simulink model "radial_fault_study_network"  (R2026b)
settings: Solver=ode23t  StopTime=0.15  MaxStep=5e-5
libraries: ee_lib x20, nesl_utility x8, simulink x5, simulink_extras x2, fl_lib x1
settings Model: Creator=ankes  LastModifiedBy=ankes
settings SimscapeCC: SimscapeLogType=all  SimscapeNominalValues="[{\"value\":\"1\",\"unit\":\"A\"},{\"value\":\"1\",\"unit\":\"bar\"},{\"value\":\"1\",\"unit\":\"cm^2\"},{\"value\":\"1\",\"unit\":\"cm^3/s\"},{\"value\":\"1\",\"unit\":\"kJ/kg\"},{\"value\":\"1\",\"unit\":\"kW\"},{\"value\":\"1\",\"unit\":\"l\"},{\"value\":\"1\",\"unit\":\"N\"},{\"value\":\"1\",\"unit\":\"N*m\"},{\"value\":\"1\",\"unit\":\"V\"},{\"value\":\"0.001\",\"unit\":\"Wb\"}]"  SimscapeUseEnergyAccounting=off

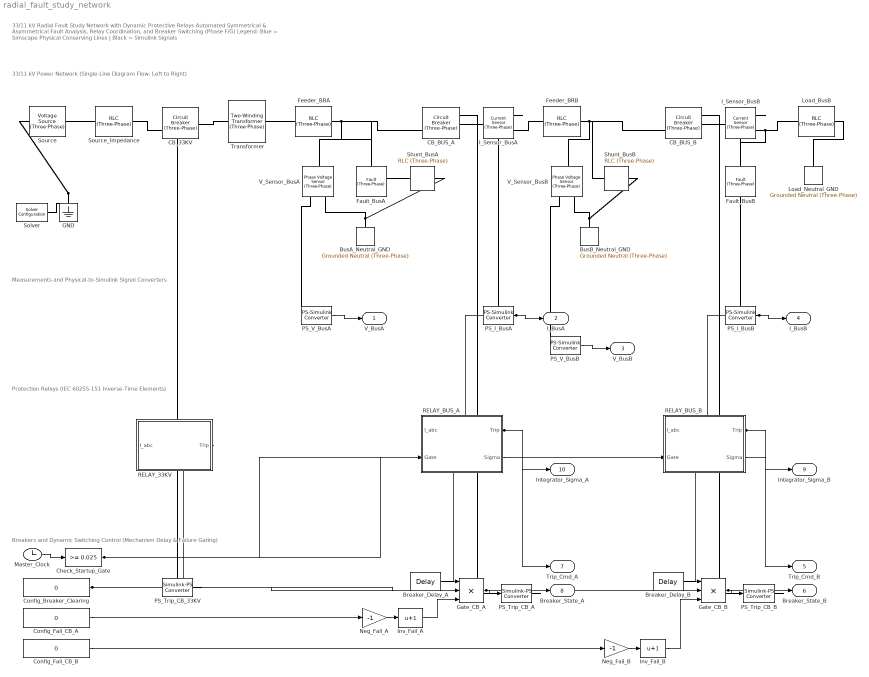
== system radial_fault_study_network ==
  note: 33/11 kV Radial Fault Study Network with Dynamic Protective Relays
      | Automated Symmetrical & Asymmetrical Fault Analysis, Relay Coordination, and Breaker Switching (Phase F/G)
      | Legend: Blue = Simscape Physical Conserving Lines  |  Black = Simulink Signals
  note: 33/11 kV Power Network (Single-Line Diagram Flow: Left to Right)
  note: Measurements and Physical-to-Simulink Signal Converters
  note: Protection Relays (IEC 60255-151 Inverse-Time Elements)
  note: Breakers and Dynamic Switching Control (Mechanism Delay & Failure Gating)
  Breaker_Delay_A : TransportDelay  DelayTime=0.06  BufferSize=8192
  Breaker_Delay_B : TransportDelay  DelayTime=0.05  BufferSize=8192
  BusA_Neutral_GND : ee_lib/Connectors & References/Grounded Neutral (Three-Phase)  port_option=ee.enum.threePhasePort.composite
  BusB_Neutral_GND : ee_lib/Connectors & References/Grounded Neutral (Three-Phase)  port_option=ee.enum.threePhasePort.composite
  CB_33KV : ee_lib/Switches & Breakers/Circuit Breaker (Three-Phase)  port_option=ee.enum.threePhasePort.composite  control_port_option=ee.enum.controlport.ps  R_closed=0.001 Ohm  G_open=1e-6 1/Ohm  threshold=0.5 V  breaker_behavior=ee.enum.switches.breakerBehavior.zeroCrossingEnable  i_th=1e-8 A
  CB_BUS_A : ee_lib/Switches & Breakers/Circuit Breaker (Three-Phase)  port_option=ee.enum.threePhasePort.composite  control_port_option=ee.enum.controlport.ps  R_closed=0.001 Ohm  G_open=1e-6 1/Ohm  threshold=0.5 V  breaker_behavior=ee.enum.switches.breakerBehavior.zeroCrossingEnable  i_th=1e-8 A
  CB_BUS_B : ee_lib/Switches & Breakers/Circuit Breaker (Three-Phase)  port_option=ee.enum.threePhasePort.composite  control_port_option=ee.enum.controlport.ps  R_closed=0.001 Ohm  G_open=1e-6 1/Ohm  threshold=0.5 V  breaker_behavior=ee.enum.switches.breakerBehavior.zeroCrossingEnable  i_th=1e-8 A
  Check_Startup_Gate : simulink/Logic and Bit Operations/Compare To Constant  relop=>=  const=0.025  OutDataTypeStr=boolean
  Config_Breaker_Clearing : Constant  Value=0
  Config_Fail_CB_A : Constant  Value=0
  Config_Fail_CB_B : Constant  Value=0
  Fault_BusA : ee_lib/Utilities/Fault (Three-Phase)  port_option=ee.enum.threePhasePort.composite  fault_type_option=ee.enum.fault_type_option.abc  R_pn_fault=0.001 Ohm  R_ng_fault=0.001 Ohm  exposemeasurement=ee.enum.exposemeasurement.hidden  enable_external_fault=ee.enum.external_fault.hidden  fault_threshold=0.5  fault_condition=ee.enum.fault_condition.fgt  fault_resettable=ee.enum.enable.no  enable_temporal_fault=ee.enum.enable.no  fault_start_time=999.0 s  fault_duration=0.20 s  G_parasitic=1e-4 1/Ohm  I_specify=off  I_priority=None  I=[0, 0, 0] A  I_nominal_specify=off  I_nominal_value=1  I_nominal_unit=A  i_ng_specify=off  i_ng_priority=None  i_ng=0 A  i_ng_nominal_specify=off  i_ng_nominal_value=1  i_ng_nominal_unit=A
  Fault_BusB : ee_lib/Utilities/Fault (Three-Phase)  port_option=ee.enum.threePhasePort.composite  fault_type_option=ee.enum.fault_type_option.abc  R_pn_fault=0.001 Ohm  R_ng_fault=0.001 Ohm  exposemeasurement=ee.enum.exposemeasurement.hidden  enable_external_fault=ee.enum.external_fault.hidden  fault_threshold=0.5  fault_condition=ee.enum.fault_condition.fgt  fault_resettable=ee.enum.enable.no  enable_temporal_fault=ee.enum.enable.yes  fault_start_time=0.05 s  fault_duration=0.20 s  G_parasitic=1e-4 1/Ohm  I_specify=off  I_priority=None  I=[0, 0, 0] A  I_nominal_specify=off  I_nominal_value=1  I_nominal_unit=A  i_ng_specify=off  i_ng_priority=None  i_ng=0 A  i_ng_nominal_specify=off  i_ng_nominal_value=1  i_ng_nominal_unit=A
  Feeder_BRA : ee_lib/Passive/RLC Assemblies/RLC (Three-Phase)  port_option=ee.enum.threePhasePort.composite  component_structure=ee.enum.rlc.structure.SeriesRL  R=0.0605 Ohm  L=0.0019258 H  C=1e-6 F  R_parasitic=0 Ohm  G_parasitic=1e-06 1/Ohm  IL_specify=off  IL_priority=High  IL=[0, 0, 0] A  IL_nominal_specify=off  IL_nominal_value=1  IL_nominal_unit=A  VC_specify=off  VC_priority=High  VC=[0, 0, 0] V  VC_nominal_specify=off  VC_nominal_value=1  VC_nominal_unit=V
  Feeder_BRB : ee_lib/Passive/RLC Assemblies/RLC (Three-Phase)  port_option=ee.enum.threePhasePort.composite  component_structure=ee.enum.rlc.structure.SeriesRL  R=0.0605 Ohm  L=0.0019258 H  C=1e-6 F  R_parasitic=0 Ohm  G_parasitic=1e-06 1/Ohm  IL_specify=off  IL_priority=High  IL=[0, 0, 0] A  IL_nominal_specify=off  IL_nominal_value=1  IL_nominal_unit=A  VC_specify=off  VC_priority=High  VC=[0, 0, 0] V  VC_nominal_specify=off  VC_nominal_value=1  VC_nominal_unit=V
  GND : fl_lib/Electrical/Electrical Elements/Electrical Reference
  Gate_CB_A : Product  Inputs=3
  Gate_CB_B : Product  Inputs=3
  I_Sensor_BusA : ee_lib/Sensors & Transducers/Current Sensor (Three-Phase)  port_option=ee.enum.threePhasePort.composite
  I_Sensor_BusB : ee_lib/Sensors & Transducers/Current Sensor (Three-Phase)  port_option=ee.enum.threePhasePort.composite
  Inv_Fail_A : Bias  Bias=1  SaturateOnIntegerOverflow=off
  Inv_Fail_B : Bias  Bias=1  SaturateOnIntegerOverflow=off
  Load_BusB : ee_lib/Passive/RLC Assemblies/RLC (Three-Phase)  port_option=ee.enum.threePhasePort.composite  component_structure=ee.enum.rlc.structure.SeriesRL  R=121 Ohm  L=0.001 H  C=1e-6 F  R_parasitic=0 Ohm  G_parasitic=0 1/Ohm  IL_specify=off  IL_priority=High  IL=[0, 0, 0] A  IL_nominal_specify=off  IL_nominal_value=1  IL_nominal_unit=A  VC_specify=off  VC_priority=High  VC=[0, 0, 0] V  VC_nominal_specify=off  VC_nominal_value=1  VC_nominal_unit=V
  Load_Neutral_GND : ee_lib/Connectors & References/Grounded Neutral (Three-Phase)  port_option=ee.enum.threePhasePort.composite
  Master_Clock : Clock
  Neg_Fail_A : Gain  Gain=-1
  Neg_Fail_B : Gain  Gain=-1
  PS_I_BusA : nesl_utility/PS-Simulink Converter  PhysicalDomain=network_engine_domain  SubClassName=ps_output  LeftPortType=input  RightPortType=output  PseudoPeriodic=off  Frequencies=[]  VectorFormat=inherit  Unit=inherit  AffineConversion=off
  PS_I_BusB : nesl_utility/PS-Simulink Converter  PhysicalDomain=network_engine_domain  SubClassName=ps_output  LeftPortType=input  RightPortType=output  PseudoPeriodic=off  Frequencies=[]  VectorFormat=inherit  Unit=inherit  AffineConversion=off
  PS_Trip_CB_33KV : nesl_utility/Simulink-PS Converter  PhysicalDomain=network_engine_domain  SubClassName=ps_input  LeftPortType=input  RightPortType=output  PseudoPeriodic=off  Frequencies=[]  NoiseDistribution=none  NoiseParameters=[]  Unit=1  AffineConversion=off  FilteringAndDerivatives=provide  SimscapeFilterOrder=1  InputFilterTimeConstant=0.001  UdotUserProvided=0
  PS_Trip_CB_A : nesl_utility/Simulink-PS Converter  PhysicalDomain=network_engine_domain  SubClassName=ps_input  LeftPortType=input  RightPortType=output  PseudoPeriodic=off  Frequencies=[]  NoiseDistribution=none  NoiseParameters=[]  Unit=1  AffineConversion=off  FilteringAndDerivatives=provide  SimscapeFilterOrder=1  InputFilterTimeConstant=0.001  UdotUserProvided=0
  PS_Trip_CB_B : nesl_utility/Simulink-PS Converter  PhysicalDomain=network_engine_domain  SubClassName=ps_input  LeftPortType=input  RightPortType=output  PseudoPeriodic=off  Frequencies=[]  NoiseDistribution=none  NoiseParameters=[]  Unit=1  AffineConversion=off  FilteringAndDerivatives=provide  SimscapeFilterOrder=1  InputFilterTimeConstant=0.001  UdotUserProvided=0
  PS_V_BusA : nesl_utility/PS-Simulink Converter  PhysicalDomain=network_engine_domain  SubClassName=ps_output  LeftPortType=input  RightPortType=output  PseudoPeriodic=off  Frequencies=[]  VectorFormat=inherit  Unit=inherit  AffineConversion=off
  PS_V_BusB : nesl_utility/PS-Simulink Converter  PhysicalDomain=network_engine_domain  SubClassName=ps_output  LeftPortType=input  RightPortType=output  PseudoPeriodic=off  Frequencies=[]  VectorFormat=inherit  Unit=inherit  AffineConversion=off
  RELAY_33KV : Subsystem
  RELAY_BUS_A : Subsystem
  RELAY_BUS_B : Subsystem
  Shunt_BusA : ee_lib/Passive/RLC Assemblies/RLC (Three-Phase)  port_option=ee.enum.threePhasePort.composite  component_structure=ee.enum.rlc.structure.R  R=100000 Ohm  L=1e-3 H  C=1e-6 F  R_parasitic=0 Ohm  G_parasitic=0 1/Ohm  IL_specify=off  IL_priority=High  IL=[0, 0, 0] A  IL_nominal_specify=off  IL_nominal_value=1  IL_nominal_unit=A  VC_specify=off  VC_priority=High  VC=[0, 0, 0] V  VC_nominal_specify=off  VC_nominal_value=1  VC_nominal_unit=V
  Shunt_BusB : ee_lib/Passive/RLC Assemblies/RLC (Three-Phase)  port_option=ee.enum.threePhasePort.composite  component_structure=ee.enum.rlc.structure.R  R=100000 Ohm  L=1e-3 H  C=1e-6 F  R_parasitic=0 Ohm  G_parasitic=0 1/Ohm  IL_specify=off  IL_priority=High  IL=[0, 0, 0] A  IL_nominal_specify=off  IL_nominal_value=1  IL_nominal_unit=A  VC_specify=off  VC_priority=High  VC=[0, 0, 0] V  VC_nominal_specify=off  VC_nominal_value=1  VC_nominal_unit=V
  Solver : nesl_utility/Solver Configuration  PhysicalDomain=network_engine_domain  SubClassName=solver  LeftPortType=input  RightPortType=generic  Tones=[]  Harmonics=[]  SimulateNoise=off  Profile=off  UseLocalSampling=off  EnableSwitchedLinearOptims=on  FrequencyDomain=off  UseCCode=off  RelTol=0.001  AbsTol=0.001  MinStep=1e-09  ToWorkspace=off  RevertToSquareIcSolve=off  NumHomotopyIterations=100  PhasorMode=off  PhasorModeNumHarmonics=1  ConsistencySolver=NEWTON_XTOL_AFTER_FTOL  CanonicalOrdering=CANONICAL  OptimizeIntermediates=OPTIMIZED  MulticoreSolverChoice=BACKWARD_EULER  IndexReductionMethod=DerivativeReplacement  DoDC=off  ResidualTolerance=1e-4  ConsistencyTolSource=GLOBAL  ConsistencyAbsTol=0.001  ConsistencyRelTol=0.001  ConsistencyTolFactor=0.001  UseLocalSolver=off  LocalSolverChoice=NE_BACKWARD_EULER_ADVANCER  ResolveIndetEquations=on  FunctionEvalNumThread=1  LocalSolverSampleTime=0.001  DoFixedCost=off  MaxNonlinIter=100  MaxModeIter=2  ComputeImpulses=off  ImpulseIterations=2  LinearAlgebra=auto  LinearAlgebraNumThread=0  EquationFormulation=NE_TIME_EF  DelaysMemoryBudget=1024  AutomaticFiltering=on  FilteringTimeConstant=0.001  PartitionStorageMethod=AS_NEEDED  PartitionMemoryBudget=1024  PartitionMethod=BALANCED  MultibodyUseLocalSolver=off  MultibodyLocalSolverChoice=ODE1  MultibodyLocalSolverSampleTime=0.001
  Source : ee_lib/Sources/Voltage Source (Three-Phase)  vline_rms=33000 V  shift=0 deg  freq=50 Hz  impedance_option=0  SShortCircuit=1e6 A*V  XR=15  R=0.01 Ohm  L=3.97e-4 H  harmonic_option=0  harmonic_orders=[5, 7, 11, 13]  harmonic_ratios=[.1, .1, .1, .1]  G_parasitic=0 1/Ohm  I_specify=off  I_priority=None  I=[0, 0, 0] A  I_nominal_specify=off  I_nominal_value=1  I_nominal_unit=A
  Source_Impedance : ee_lib/Passive/RLC Assemblies/RLC (Three-Phase)  port_option=ee.enum.threePhasePort.composite  component_structure=ee.enum.rlc.structure.SeriesRL  R=0.1089 Ohm  L=0.034665 H  C=1e-6 F  R_parasitic=0 Ohm  G_parasitic=1e-06 1/Ohm  IL_specify=off  IL_priority=High  IL=[0, 0, 0] A  IL_nominal_specify=off  IL_nominal_value=1  IL_nominal_unit=A  VC_specify=off  VC_priority=High  VC=[0, 0, 0] V  VC_nominal_specify=off  VC_nominal_value=1  VC_nominal_unit=V
  Transformer : ee_lib/Passive/Transformers/Two-Winding Transformer (Three-Phase)  port_option=ee.enum.threePhasePort.composite  SRated=10000000 A*V  FRated=50 Hz  Winding1Connection=ee.enum.windingconnection.Yg  VRated1=33000 V  Winding2Connection=ee.enum.windingconnection.Yg  VRated2=11000 V  param_option=ee.enum.transformer_parameterization.circuitimpedances  CoreType=ee.enum.coretype.threelimb  pu_Rw1=0.002  pu_Rw2=0.002  leakage_reactance_option=ee.enum.transformer_leakage.include  pu_Xl1=0.04  pu_Xl2=0.04  magnetizing_resistance_option=ee.enum.transformer_magnetizingResistance.exclude  pu_Rm=500  magnetizing_reactance_option=ee.enum.transformer_magnetizingReactance.exclude  saturation_option=ee.enum.transformer_saturation.exclude  pu_Xm=500  current_data=[0, .002, 1, 2]  magnetic_flux_data=[0, 1.2, 1.5, 1.51]  pu_X0=0.5  pu_Rw1_td=0.01  pu_Rw2_td=0.01  pu_X121=0.1  pu_P1=0.01  pu_Iext1=0.02  zero_sequence_data=ee.enum.transformer_zeroSequence.exclude  pu_X120=0.09  pu_P0=0.15  pu_Iext0=3.5  saturation_option_td=ee.enum.transformer_saturation.exclude  current_data_td=[0, .002, 1, 2]  magnetic_flux_data_td=[0, 1.2, 1.5, 1.51]  i1_specify=off  i1_priority=None  i1=[0, 0, 0] A  i1_nominal_specify=off  i1_nominal_value=1  i1_nominal_unit=A  i2_specify=off  i2_priority=None  i2=[0, 0, 0] A  i2_nominal_specify=off  i2_nominal_value=1  i2_nominal_unit=A  phi_specify=off  phi_priority=None  phi=[0, 0, 0]  phi_nominal_specify=off  phi_nominal_value=1  phi_nominal_unit=1
  V_Sensor_BusA : ee_lib/Sensors & Transducers/Phase Voltage Sensor (Three-Phase)  port_option=ee.enum.threePhasePort.composite
  V_Sensor_BusB : ee_lib/Sensors & Transducers/Phase Voltage Sensor (Three-Phase)  port_option=ee.enum.threePhasePort.composite
  V_BusA : Outport
  I_BusA : Outport  Port=2
  V_BusB : Outport  Port=3
  I_BusB : Outport  Port=4
  Trip_Cmd_B : Outport  Port=5
  Breaker_State_B : Outport  Port=6
  Trip_Cmd_A : Outport  Port=7
  Breaker_State_A : Outport  Port=8
  Integrator_Sigma_B : Outport  Port=9
  Integrator_Sigma_A : Outport  Port=10
  wires:
  PS_V_BusA/1 -> V_BusA/1
  PS_I_BusA/1 -> I_BusA/1, RELAY_BUS_A/1(I_abc)
  PS_V_BusB/1 -> V_BusB/1
  PS_I_BusB/1 -> I_BusB/1, RELAY_BUS_B/1(I_abc)
  Master_Clock/1 -> Check_Startup_Gate/1
  RELAY_33KV/1(Trip) -> PS_Trip_CB_33KV/1
  Check_Startup_Gate/1 -> RELAY_BUS_A/2(Gate), RELAY_BUS_B/2(Gate)
  RELAY_BUS_A/2(Sigma) -> Integrator_Sigma_A/1
  RELAY_BUS_A/1(Trip) -> Trip_Cmd_A/1, Breaker_Delay_A/1
  Breaker_Delay_A/1 -> Gate_CB_A/1
  Config_Breaker_Clearing/1 -> Gate_CB_A/2, Gate_CB_B/2
  Config_Fail_CB_A/1 -> Neg_Fail_A/1
  Neg_Fail_A/1 -> Inv_Fail_A/1
  Inv_Fail_A/1 -> Gate_CB_A/3
  Gate_CB_A/1 -> Breaker_State_A/1, PS_Trip_CB_A/1
  RELAY_BUS_B/2(Sigma) -> Integrator_Sigma_B/1
  RELAY_BUS_B/1(Trip) -> Trip_Cmd_B/1, Breaker_Delay_B/1
  Breaker_Delay_B/1 -> Gate_CB_B/1
  Config_Fail_CB_B/1 -> Neg_Fail_B/1
  Neg_Fail_B/1 -> Inv_Fail_B/1
  Inv_Fail_B/1 -> Gate_CB_B/3
  Gate_CB_B/1 -> Breaker_State_B/1, PS_Trip_CB_B/1
  connections:
  GND/LConn1 -- Solver/RConn1 -- Source/LConn1
  Source/RConn1 -- Source_Impedance/LConn1
  Source_Impedance/RConn1 -- CB_33KV/LConn2
  CB_33KV/RConn1 -- Transformer/LConn1
  Transformer/RConn1 -- Feeder_BRA/LConn1
  V_Sensor_BusA/LConn1 -- Feeder_BRA/RConn1 -- Shunt_BusA/LConn1 -- Fault_BusA/LConn1 -- CB_BUS_A/LConn2
  BusA_Neutral_GND/LConn1 -- V_Sensor_BusA/RConn2 -- Shunt_BusA/RConn1
  CB_BUS_A/RConn1 -- I_Sensor_BusA/LConn1
  I_Sensor_BusA/RConn2 -- Feeder_BRB/LConn1
  V_Sensor_BusB/LConn1 -- Feeder_BRB/RConn1 -- Shunt_BusB/LConn1 -- CB_BUS_B/LConn2
  BusB_Neutral_GND/LConn1 -- V_Sensor_BusB/RConn2 -- Shunt_BusB/RConn1
  CB_BUS_B/RConn1 -- I_Sensor_BusB/LConn1
  Load_BusB/LConn1 -- I_Sensor_BusB/RConn2 -- Fault_BusB/LConn1
  Load_BusB/RConn1 -- Load_Neutral_GND/LConn1
  V_Sensor_BusA/RConn1 -- PS_V_BusA/LConn1
  I_Sensor_BusA/RConn1 -- PS_I_BusA/LConn1
  V_Sensor_BusB/RConn1 -- PS_V_BusB/LConn1
  I_Sensor_BusB/RConn1 -- PS_I_BusB/LConn1
  PS_Trip_CB_33KV/RConn1 -- CB_33KV/LConn1
  PS_Trip_CB_A/RConn1 -- CB_BUS_A/LConn1
  PS_Trip_CB_B/RConn1 -- CB_BUS_B/LConn1

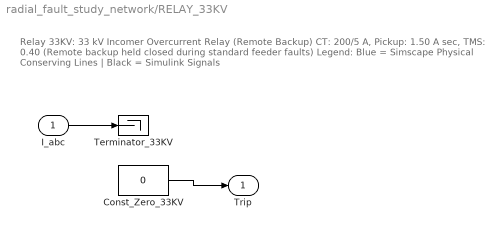
== system radial_fault_study_network/RELAY_33KV ==
  note: Relay 33KV: 33 kV Incomer Overcurrent Relay (Remote Backup)
      | CT: 200/5 A, Pickup: 1.50 A sec, TMS: 0.40 (Remote backup held closed during standard feeder faults)
      | Legend: Blue = Simscape Physical Conserving Lines  |  Black = Simulink Signals
  I_abc : Inport
  Const_Zero_33KV : Constant  Value=0
  Terminator_33KV : Terminator
  Trip : Outport
  wires:
  I_abc/1 -> Terminator_33KV/1
  Const_Zero_33KV/1 -> Trip/1

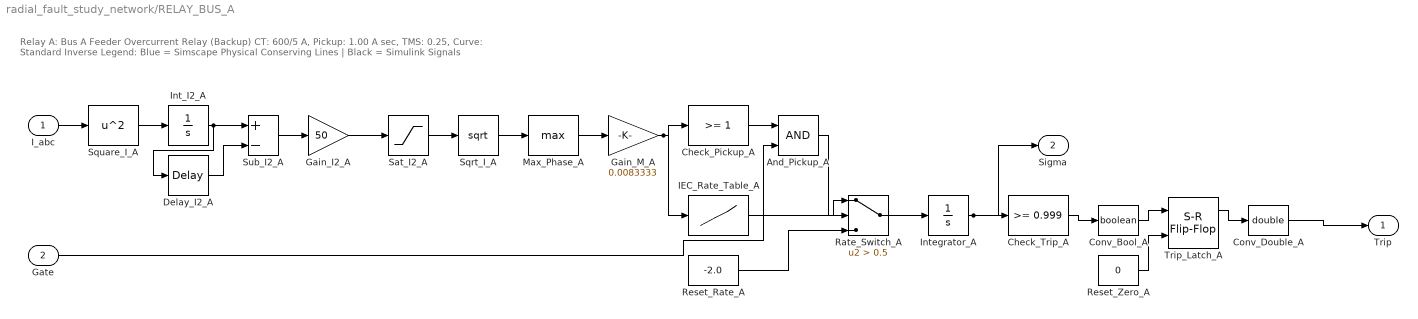
== system radial_fault_study_network/RELAY_BUS_A ==
  note: Relay A: Bus A Feeder Overcurrent Relay (Backup)
      | CT: 600/5 A, Pickup: 1.00 A sec, TMS: 0.25, Curve: Standard Inverse
      | Legend: Blue = Simscape Physical Conserving Lines  |  Black = Simulink Signals
  I_abc : Inport
  Gate : Inport  Port=2
  And_Pickup_A : Logic  AllPortsSameDT=off  OutDataTypeStr=boolean
  Check_Pickup_A : simulink/Logic and Bit Operations/Compare To Constant  relop=>=  const=1  OutDataTypeStr=boolean
  Check_Trip_A : simulink/Logic and Bit Operations/Compare To Constant  relop=>=  const=0.999  OutDataTypeStr=boolean
  Conv_Bool_A : DataTypeConversion  OutDataTypeStr=boolean  SaturateOnIntegerOverflow=off  RndMeth=Floor
  Conv_Double_A : DataTypeConversion  OutDataTypeStr=double  SaturateOnIntegerOverflow=off  RndMeth=Floor
  Delay_I2_A : TransportDelay  DelayTime=0.020  BufferSize=8192
  Gain_I2_A : Gain  Gain=50
  Gain_M_A : Gain  Gain=0.0083333
  IEC_Rate_Table_A : Lookup_n-D  NumberOfTableDimensions=1  BreakpointsForDimension1=[1 1.005 1.01 1.02 1.05 1.1 1.2 1.5 2 3 5 10 20 30 50 100]  Table=[0 0.00285 0.00569 0.01132 0.02789 0.05451 0.10437 0.23264 0.39884 0.63473 0.93464 1.34653 1.76417 2.01117 2.32522 2.75652]  InternalRulePriority=Speed  RndMeth=Simplest
  Int_I2_A : Integrator
  Integrator_A : Integrator  LimitOutput=on  UpperSaturationLimit=1.0  LowerSaturationLimit=0.0
  Max_Phase_A : MinMax  Function=max
  Rate_Switch_A : Switch  Criteria=u2 > Threshold  Threshold=0.5  SaturateOnIntegerOverflow=off  InputSameDT=off
  Reset_Rate_A : Constant  Value=-2.0
  Reset_Zero_A : Constant  Value=0  OutDataTypeStr=boolean
  Sat_I2_A : Saturate  UpperLimit=inf  LowerLimit=0
  Sqrt_I_A : Sqrt
  Square_I_A : Math  Operator=square
  Sub_I2_A : Sum  Inputs=+-
  Trip_Latch_A : simulink_extras/Flip Flops/S-R Flip-Flop  initial_condition=0
  Trip : Outport
  Sigma : Outport  Port=2
  wires:
  I_abc/1 -> Square_I_A/1
  Square_I_A/1 -> Int_I2_A/1
  Int_I2_A/1 -> Delay_I2_A/1, Sub_I2_A/1
  Delay_I2_A/1 -> Sub_I2_A/2
  Sub_I2_A/1 -> Gain_I2_A/1
  Gain_I2_A/1 -> Sat_I2_A/1
  Sat_I2_A/1 -> Sqrt_I_A/1
  Sqrt_I_A/1 -> Max_Phase_A/1
  Max_Phase_A/1 -> Gain_M_A/1
  Gain_M_A/1 -> Check_Pickup_A/1, IEC_Rate_Table_A/1
  Check_Pickup_A/1 -> And_Pickup_A/1
  Gate/1 -> And_Pickup_A/2
  IEC_Rate_Table_A/1 -> Rate_Switch_A/1
  And_Pickup_A/1 -> Rate_Switch_A/2
  Reset_Rate_A/1 -> Rate_Switch_A/3
  Rate_Switch_A/1 -> Integrator_A/1
  Integrator_A/1 -> Sigma/1, Check_Trip_A/1
  Check_Trip_A/1 -> Conv_Bool_A/1
  Conv_Bool_A/1 -> Trip_Latch_A/1
  Reset_Zero_A/1 -> Trip_Latch_A/2
  Trip_Latch_A/1 -> Conv_Double_A/1
  Conv_Double_A/1 -> Trip/1

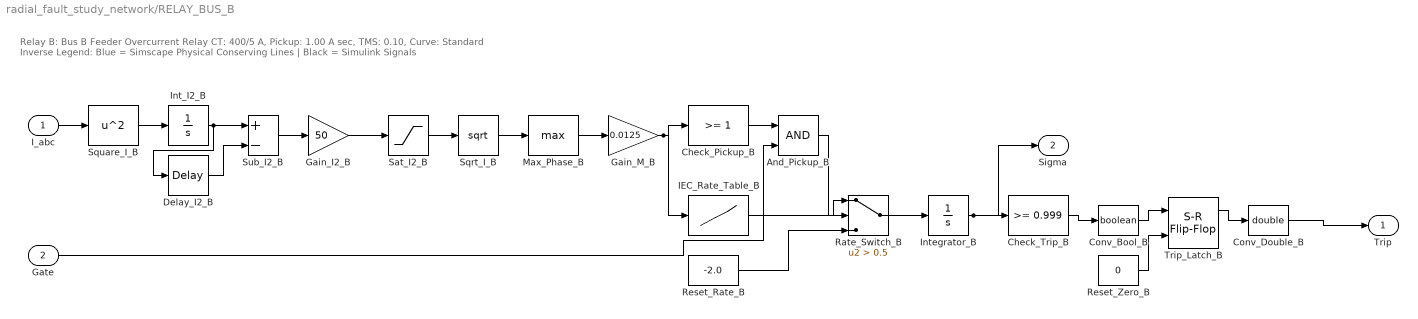
== system radial_fault_study_network/RELAY_BUS_B ==
  note: Relay B: Bus B Feeder Overcurrent Relay
      | CT: 400/5 A, Pickup: 1.00 A sec, TMS: 0.10, Curve: Standard Inverse
      | Legend: Blue = Simscape Physical Conserving Lines  |  Black = Simulink Signals
  I_abc : Inport
  Gate : Inport  Port=2
  And_Pickup_B : Logic  AllPortsSameDT=off  OutDataTypeStr=boolean
  Check_Pickup_B : simulink/Logic and Bit Operations/Compare To Constant  relop=>=  const=1  OutDataTypeStr=boolean
  Check_Trip_B : simulink/Logic and Bit Operations/Compare To Constant  relop=>=  const=0.999  OutDataTypeStr=boolean
  Conv_Bool_B : DataTypeConversion  OutDataTypeStr=boolean  SaturateOnIntegerOverflow=off  RndMeth=Floor
  Conv_Double_B : DataTypeConversion  OutDataTypeStr=double  SaturateOnIntegerOverflow=off  RndMeth=Floor
  Delay_I2_B : TransportDelay  DelayTime=0.020  BufferSize=8192
  Gain_I2_B : Gain  Gain=50
  Gain_M_B : Gain  Gain=0.0125
  IEC_Rate_Table_B : Lookup_n-D  NumberOfTableDimensions=1  BreakpointsForDimension1=[1 1.005 1.01 1.02 1.05 1.1 1.2 1.5 2 3 5 10 20 30 50 100]  Table=[0 0.00713 0.01422 0.0283 0.06973 0.13629 0.26093 0.58159 0.99711 1.58682 2.3366 3.36632 4.41042 5.02792 5.81305 6.8913]  InternalRulePriority=Speed  RndMeth=Simplest
  Int_I2_B : Integrator
  Integrator_B : Integrator  LimitOutput=on  UpperSaturationLimit=1.0  LowerSaturationLimit=0.0
  Max_Phase_B : MinMax  Function=max
  Rate_Switch_B : Switch  Criteria=u2 > Threshold  Threshold=0.5  SaturateOnIntegerOverflow=off  InputSameDT=off
  Reset_Rate_B : Constant  Value=-2.0
  Reset_Zero_B : Constant  Value=0  OutDataTypeStr=boolean
  Sat_I2_B : Saturate  UpperLimit=inf  LowerLimit=0
  Sqrt_I_B : Sqrt
  Square_I_B : Math  Operator=square
  Sub_I2_B : Sum  Inputs=+-
  Trip_Latch_B : simulink_extras/Flip Flops/S-R Flip-Flop  initial_condition=0
  Trip : Outport
  Sigma : Outport  Port=2
  wires:
  I_abc/1 -> Square_I_B/1
  Square_I_B/1 -> Int_I2_B/1
  Int_I2_B/1 -> Delay_I2_B/1, Sub_I2_B/1
  Delay_I2_B/1 -> Sub_I2_B/2
  Sub_I2_B/1 -> Gain_I2_B/1
  Gain_I2_B/1 -> Sat_I2_B/1
  Sat_I2_B/1 -> Sqrt_I_B/1
  Sqrt_I_B/1 -> Max_Phase_B/1
  Max_Phase_B/1 -> Gain_M_B/1
  Gain_M_B/1 -> Check_Pickup_B/1, IEC_Rate_Table_B/1
  Check_Pickup_B/1 -> And_Pickup_B/1
  Gate/1 -> And_Pickup_B/2
  IEC_Rate_Table_B/1 -> Rate_Switch_B/1
  And_Pickup_B/1 -> Rate_Switch_B/2
  Reset_Rate_B/1 -> Rate_Switch_B/3
  Rate_Switch_B/1 -> Integrator_B/1
  Integrator_B/1 -> Sigma/1, Check_Trip_B/1
  Check_Trip_B/1 -> Conv_Bool_B/1
  Conv_Bool_B/1 -> Trip_Latch_B/1
  Reset_Zero_B/1 -> Trip_Latch_B/2
  Trip_Latch_B/1 -> Conv_Double_B/1
  Conv_Double_B/1 -> Trip/1
